simulink subsystem "R2Geodetic"  (R2024b)
settings: Solver=VariableStepAuto  StartTime=0.0  StopTime=10.0  RelTol=1e-3
settings Model: Creator=marco  LastModifiedBy=ferru

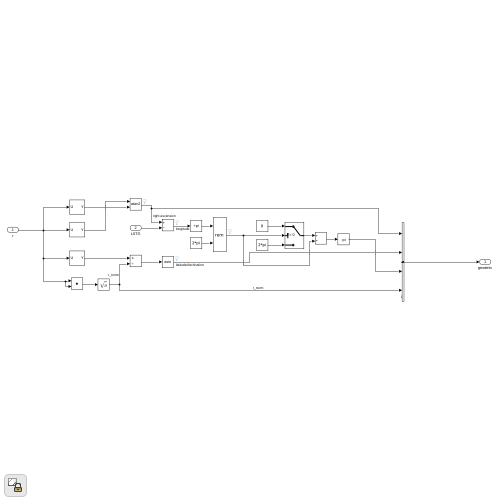
[thumbnail: Simulink's stored preview of the top-level diagram]
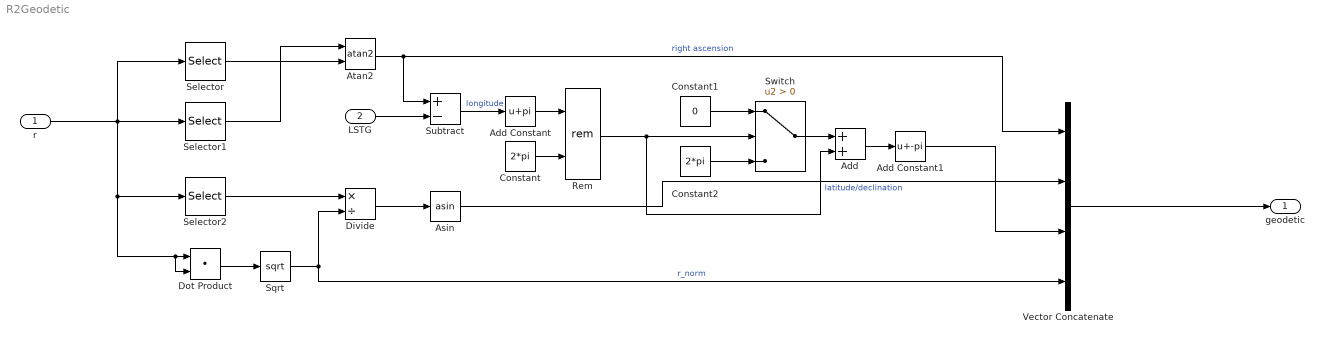
== system R2Geodetic ==
  r : Inport
  LSTG : Inport  Port=2
  Add : Sum
  Add Constant : Bias  Bias=pi  SaturateOnIntegerOverflow=off
  Add Constant1 : Bias  Bias=-pi  SaturateOnIntegerOverflow=off
  Asin : Trigonometry  Operator=asin
  Atan2 : Trigonometry  Operator=atan2
  Constant : Constant  Value=2*pi
  Constant1 : Constant  Value=0
  Constant2 : Constant  Value=2*pi
  Divide : Product  Inputs=*/
  Dot Product : DotProduct  OutDataTypeStr=Inherit: Inherit via internal rule
  Rem : Math  Operator=rem
  Selector : Selector  NumberOfDimensions=2  InputPortWidth=3  IndexOptions=Index vector (dialog),Select all  Indices=1,1  OutputSizes=1,1
  Selector1 : Selector  NumberOfDimensions=2  InputPortWidth=3  IndexOptions=Index vector (dialog),Select all  Indices=2,1  OutputSizes=1,1
  Selector2 : Selector  NumberOfDimensions=2  InputPortWidth=3  IndexOptions=Index vector (dialog),Select all  Indices=3,1  OutputSizes=1,1
  Sqrt : Sqrt
  Subtract : Sum  Inputs=+-
  Switch : Switch  Criteria=u2 > Threshold  SaturateOnIntegerOverflow=off  InputSameDT=off
  Vector Concatenate : Concatenate  NumInputs=4  Mode=Multidimensional array
  geodetic : Outport
  wires:
  r/1 -> Selector1/1, Selector2/1, Dot Product/1, Dot Product/2, Selector/1
  Selector1/1 -> Atan2/1
  Selector/1 -> Atan2/2
  Dot Product/1 -> Sqrt/1
  Selector2/1 -> Divide/1
  Sqrt/1 -> Vector Concatenate/4, Divide/2  "r_norm"
  Divide/1 -> Asin/1
  Atan2/1 -> Vector Concatenate/1, Subtract/1  "right ascension"
  LSTG/1 -> Subtract/2
  Subtract/1 -> Add Constant/1  "longitude"
  Asin/1 -> Vector Concatenate/2  "latitude/declination"
  Vector Concatenate/1 -> geodetic/1
  Constant/1 -> Rem/2
  Rem/1 -> Switch/2, Add/2
  Add Constant/1 -> Rem/1
  Constant1/1 -> Switch/1
  Constant2/1 -> Switch/3
  Switch/1 -> Add/1
  Add/1 -> Add Constant1/1
  Add Constant1/1 -> Vector Concatenate/3
